simulink model "ball_impact"  (Simulink 8.1)
settings: Solver=ode4  SolverMode=SingleTasking  StartTime=0.0  StopTime=inf  FixedStep=0.0005  RelTol=1e-3
StartFcn:
  |  warndlg('Dexterit-E models cannot run under simulation. Please compile your model and run it from within Dexterit-E.');set_param(bdroot,'SimulationCommand','stop')
undefined symbols (not defined in the file or in its folder): CreateParameterTableGUI, slselsubs
libraries: xpclib x30, simulink x8, KINARM_general x3, KINARM_loads x2, Video x2, KINARM_EP_loads x1
(part 5 of 5)

== matlab function DataLogging/Receive_Gaze/Embedded MATLAB Function1 ==
  data: input input double; pupil_area_PIXELS input double; tracking_status input double; tracking_available input double; camtheta input double; camera_GLOBAL input double; focal_length input double; gazeXYCalculated output double; target_distance_in input double; pupil_area_GLOBAL output double
function [gazeXYCalculated, pupil_area_GLOBAL] = fcn(input, pupil_area_PIXELS, tracking_status, tracking_available, camtheta,camera_GLOBAL, focal_length, target_distance_in)

% The following are some details on the Eyelink camera
EL_target_distance_scaling_factor = 10000;					%target distance is reported by Eyelink in 1/10 of mm units
EL_pix_per_mm = 200;										%there are 200 pixels/mm on the Eyelink 1000 camera sensor

raw_pupil = [input(1) input(2)];
href = [input(3); input(4); 0];
target_distance = target_distance_in / EL_target_distance_scaling_factor;		% distance of the target from the camera (m)

%if there is a blink or other problem then send out errors. C3D file does not like NaN, so we output -100.
if tracking_status == 4 || tracking_available == 0 || (href(1) == 0 && href(2) == 0) || (raw_pupil(1) == -32768 && raw_pupil(2) == -32768)
    gazeXYCalculated = [-100; -100];
	pupil_area_GLOBAL = -100;
% % % 	testing = [0 0 0 0 0 0];
% % % 	testing2 = [0; 0; 0; 0; 0; 0];
    return
end

[Rx Ry Rz] = calc_R_from_angles(camtheta(1), camtheta(2), 0);
R_CMRA2GLBL = Rx * Ry;
%R_GLBL2CMRA = R_CMRA2GLBL';

%camera_GLOBAL_Trans = camera_GLOBAL';
pupil_XY_Sensor = convertPupilToSensor(raw_pupil(1), raw_pupil(2), EL_pix_per_mm);
[gaze_GLOBAL, pupil_GLOBAL] = calc_GAZE(pupil_XY_Sensor, target_distance, href, focal_length, camera_GLOBAL, R_CMRA2GLBL);
gazeXYCalculated = gaze_GLOBAL(1:2);

%%convert the pupil area from pixels on the sensor, to m^2, correcting for camera and gaze angle
% pupil area on the camera sensor, in m^2
pupil_area_SENSOR = pupil_area_PIXELS / ( (EL_pix_per_mm * 1000 ) ^ 2);		

% pupil area in the global workspace, projected onto a plane parallel to the camera sensor in m^2
pupil_area_GLOBAL_projection = pupil_area_SENSOR * (target_distance / focal_length) ^ 2; 

% create a unit vector that is normal to the camera sensor, in GLOBAL coordinates
sensor_unit_vector_GLOBAL = R_CMRA2GLBL * [0; 0; 1];

% create a unit vector for the subject's gaze
gaze_vector_GLOBAL = pupil_GLOBAL - gaze_GLOBAL;
gaze_unit_vector_GLOBAL = gaze_vector_GLOBAL / norm(gaze_vector_GLOBAL);

% calculate the cosine of the angle between the unit vectors for gaze and the camera sensor
cos_gaze_camera_angle = dot(sensor_unit_vector_GLOBAL, gaze_unit_vector_GLOBAL); 

% correct the pupil area to account for the angle of the eye relative to the camera sensor plane
% We assume that the pupil is circular. In the plane formed by the two vectors, the distance needs 
% to be scaled by cos(theta). In the perpendicular plane, there is no scaling. Hence we do NOT 
% square the cos(theta) and the area is only corrected for by 1 / cos(theta). 
pupil_area_GLOBAL = pupil_area_GLOBAL_projection / cos_gaze_camera_angle;

% % % % For testing
% % % gaze_camera_angle  = acos(cos_gaze_camera_angle) * 180/pi();
% % % HREF_angle = atan2( norm(href), 15000) * 180 / pi();
% % % testing = [pupil_area_SENSOR*1e6, pupil_area_GLOBAL_projection*1e6, pupil_area_GLOBAL*1e6, gaze_camera_angle, HREF_angle, cos_gaze_camera_angle];
% % % testing2 = [sensor_unit_vector_GLOBAL; gaze_unit_vector_GLOBAL];



%% Functions
function [gaze_est_GLOBAL, pupil_GLOBAL] = calc_GAZE(pupil_SENSOR, target_distance, HREF_HREF, focal_length, camera_GLOBAL, R_CMRA2GLBL)
    % This function estimates GAZE based on data from the Eyelink.  To be used
    % during 'running' of a task. 

    % Convert pupil location from Eyelink sensor frame to camera reference
    % frame with camera at origin and rotated to camera's angle (W-axis along
    % camera's point of view)  
    pupil_CAMERA = [pupil_SENSOR * target_distance / focal_length; target_distance];
    pupil_distance = norm(pupil_CAMERA);

    % Rotation matrix to convert from HREF coordinates to camera coordinates.
    % HREF z-axis is defined as ray from camera to pupil.
    R_HREF2CMRA = calc_R_from_vectors(pupil_CAMERA, [0; 0; 1]);

    % Convert the HREF from HREF coordinates to canera coordinates.  Scale,
    % then rotate. 
    HREF_CAMERA = R_HREF2CMRA * (HREF_HREF * pupil_distance / 15000);

    % Then convert pupil and HREF locations from camera frame to global frame
    % by rotating and then shifting origins. 
    pupil_GLOBAL = R_CMRA2GLBL * pupil_CAMERA + camera_GLOBAL';
    HREF_GLOBAL = R_CMRA2GLBL * HREF_CAMERA + camera_GLOBAL';

    % Find intersection of gaze_ray (from pupil to HREF) with the subject_display plane
    norm_vector = [0; 0; 1];		% In the KINARM VR setup, the Z-axis is defined as normal to the subject display
    point_on_plane = [0; 0; 0];		% In the KINARM VR setup, the origin is defined as on the subject display plane

    % display([pupil_GLOBAL HREF_GLOBAL])
    gaze_est_GLOBAL = plane_line_intersect(norm_vector, point_on_plane, pupil_GLOBAL, HREF_GLOBAL);

function pupil_XY_Sensor = convertPupilToSensor(pupilX, pupilY, pix_per_mm)
%         Returns the projection of the pupil on the camera sensor in meters, based on inputs in some raw unit (not pixels)

    % the following constants are from Jiye, email Nov 7, 2011
    LEFTDROP = 32;				%pixels dropped at left of sensor
    TOPDROP = 48;				%lines dropped at top of sensor
    const_x = 7*176;			%no idea what this is.  Maybe number of pixels???
    const_y = 4*184 + 188;		%no idea what this is.  Maybe number of pixels???

    % from Jiye. Not sure excatly what they are (probably camera center in pixels)
    cam_rot_cx = const_x / 2 + LEFTDROP;			
    cam_rot_cy = const_y / 2 +TOPDROP;

    hor = 30000;
    lor = -30000;
    hr = 0.9;
    lr = 0.1;
    ld = 50;
    hdx = 1200;		%hmmm almost same as const_x, which is 1232
    hdy = 920;		%hmmm almost same as const_y, which is 924

    scx = (hor-lor) / (hdx - ld) / (hr-lr);
    ofx = lor - (ld + (hdx - ld) * lr )* scx;

    scy = (hor-lor) / (hdy - ld) / (hr-lr);
    ofy = lor - (ld + (hdy - ld) * lr )* scy;

    % calculate the pupil in camera sensor coordinates (pixels)
    px = (pupilX - ofx) / scx;
    py = (pupilY - ofy) / scy;

    ppl_mmX = - ( (cam_rot_cx - px) / pix_per_mm );
    ppl_mmY =   ( (cam_rot_cy - py) / pix_per_mm );

    pupil_XY_Sensor = [ppl_mmX / 1000; ppl_mmY / 1000];
    
function [Rx Ry Rz] = calc_R_from_angles(xrot, yrot, zrot)
    % This function creates the three rotation matrices for rotations about the
    % x, y and z axes.  Input rotations are in degrees.

    xrot = xrot/180*pi;		%convert to radians
    yrot = yrot/180*pi;		%convert to radians
    zrot = zrot/180*pi;		%convert to radians
    Rx = [1 0 0; 0 cos(xrot) -sin(xrot); 0 sin(xrot) cos(xrot)]; 
    Ry = [cos(yrot) 0 sin(yrot); 0 1 0; -sin(yrot) 0 cos(yrot)]; 
    Rz = [cos(zrot) -sin(zrot) 0; sin(zrot) cos(zrot) 0 ; 0 0 1]; 

    
function R = calc_R_from_vectors(v1, v2)
    % This function calculates a rotation matrix, given two vectors, such that
    % the rotation matrix will rotate from v1 to v2.

    rot_axis = cross(v2, v1);			%axis that is perpendicular to the two vectors

    % If either of the vectors v1 or v2 is = [0 0 0], or if they are parallel
    % (i.e. norm(rot_axis) == 0), then there is no rotation.  But math errors
    % will occur, so we need to check for these cases.   
    if (norm(v1) == 0) || (norm(v2) == 0)	|| (norm(rot_axis) == 0)
        R = eye(3);																%identity matrix results in no rotation
    else
        rot_angle = asin( norm(rot_axis) / norm(v1) / norm(v2) );				%angle of rotation about rot_axis
        n = rot_axis / norm(rot_axis);											%normalize to get a unit vector for the rotation
        n_cross_product_matrix = [ 0 -n(3) n(2); n(3) 0 -n(1); -n(2) n(1) 0];	%def'n of cross product matrix
        cosA = cos(rot_angle);
        sinA = sin(rot_angle);
        R = eye(3) * cosA + sinA * n_cross_product_matrix + (1 - cosA) * (n * n');
    % 	display(rot_angle);
    end


function I = plane_line_intersect(n,V0,P0,P1)
    %plane_line_intersect computes the intersection of a plane and a segment(or
    %a straight line)
    % Inputs: 
    %       n: normal vector of the Plane 
    %       V0: any point that belongs to the Plane 
    %       P0: end point 1 of the segment P0P1
    %       P1:  end point 2 of the segment P0P1
    %
    %Outputs:
    %      I    is the point of interection 
    %     Check is (DELETED AND NOT USED HERE) an indicator:
    %      0 => disjoint (no intersection)
    %      1 => the plane intersects P0P1 in the unique point I
    %      2 => the segment lies in the plane
    %      3=>the intersection lies outside the segment P0P1
    %
    % Example:
    % Determine the intersection of following the plane x+y+z+3=0 with the segment P0P1:
    % The plane is represented by the normal vector n=[1 1 1]
    % and an arbitrary point that lies on the plane, ex: V0=[1 1 -5]
    % The segment is represented by the following two points
    % P0=[-5 1 -1]
    %P1=[1 2 3]   
    % [I,check]=plane_line_intersect([1 1 1],[1 1 -5],[-5 1 -1],[1 2 3]);

    %This function is written by :
    %                             Nassim Khaled
    %                             Wayne State University
    %                             Research Assistant and Phd candidate
    %If you have any comments or face any problems, please feel free to leave
    %your comments and i will try to reply to you as fast as possible.

    I=[0; 0; 0];
    u = P1-P0;
    w = P0 - V0;
    D = dot(n,u);
    N = -dot(n,w);
    check=0;
    if abs(D) < 10^-7        % The segment is parallel to plane
            if N == 0           % The segment lies in plane
                check=2;
                return
            else
                check=0;       %no intersection
                return
            end
    end

    %compute the intersection parameter
    sI = N / D;
    I = P0+ sI.*u;

== matlab function DataLogging/Receive_Gaze/clean_packet ==
  data: pack_in input double; pack_out output double; len_out output double; len_in input double
function [pack_out, len_out] = clean_packet(pack_in, len_in)

%for some reason, during calibration we can get very large packets that 
%blow up the c code for parsing the packets. If we get a large packet
%we can ignore it.

if len_in < 512
    pack_out = pack_in;
    len_out = len_in;
else
    pack_out = zeros(512, 1, 'uint8');
    len_out = int32(0);
end

== matlab function DataLogging/Receive_Gaze/convert to seconds ==
  data: event_data input double; event_data_out output double; start_time input double
function event_data_out = fcn(event_data, start_time)

event_data_out = event_data;

if event_data(1) ~= 0
    event_data_out(2) = (event_data(2) - start_time) / 1000.0;
    event_data_out(3) = (event_data(3) - start_time) / 1000.0;
end

== matlab function DataLogging/Poll Force Plates/plate2/parse packet 1 ==
  data: packet input double; forces output double; moments output double; timer output double; calibration input double; gain input double; ain_slope input double; ain_offset input double; orientation input double; zero_voltage input double
function [forces, moments, timer] = fcn(packet, calibration, gain, ain_slope, ain_offset, orientation, zero_voltage)
    %This pulls voltages and timer infomation from the packet we got back from
    %the lab jack.
    
    voltages = zeros(1, 8);
    timers = zeros(1, 3);

    for n = 1:8
        bits = readUShort(packet, 13 + ((n - 1)*2));
        voltages(n) = binaryToCalibratedAnalogVoltage(bits, ain_slope, ain_offset);
    end
    
    for n = 1:3
        timers(n) = readUInt(packet, 53 + ((n - 1)*4));
    end
    
    %convert the time stamp to a time in seconds.
    timer = timers(1) / 750000.0; 
    
    %all voltages are between -2.5 to 2.5, here we are normalizeing what we read to zero.
    voltages = voltages - zero_voltage;
    voltages = voltages(1:8); % only the first 8 channels matter.
    
    %using the calibration matrix we convert the to the forces and moments
    values = calibration * (voltages / gain)';
    forces = values(1:3);
    moments = values(4:6);
    
	%reverse the Z force to get it into global coordinates.
	forces(3) = -forces(3);

	%considering the positions of the cables push all measures into global coordinates
    if orientation == 0
        forces(2) = -forces(2);
        moments(2) = -moments(2);
    elseif orientation == 90
        y = forces(2);
        forces(2) = -forces(1);
        forces(1) = -y;

        y = moments(2);
        moments(2) = -moments(1);
        moments(1) = -y;
	elseif orientation == 180
        forces(1) = -forces(1);        
        moments(1) = -moments(1);        
    elseif orientation == 270
        y = forces(2);
        forces(2) = forces(1);
        forces(1) = y;

		y = moments(2);
        moments(2) = moments(1);
        moments(1) = y;
    end
end

function val = readUShort(data, offset)
    p1 = uint32(data(offset));
    p2 = uint32(data(offset + 1));
    val = double(p1 + (p2 * 256));
end

function val = readUInt(data, offset)
    p1 = uint32(data(offset));
    p2 = uint32(data(offset + 1));
    p3 = uint32(data(offset + 2));
    p4 = uint32(data(offset + 3));
    val = double(p1 + (p2 * 256) + (p3 * 2^16) + (p4 * 2^24));
end

function voltage = binaryToCalibratedAnalogVoltage(bits, ain_slope, ain_offset)
    voltage = (bits * ain_slope) + ain_offset;
end
